simulink model "Sistemas"  (R2020b)
settings: Solver=ode15s  StartTime=0.0  StopTime=10  MaxStep=1E-2  RelTol=1e-3
libraries: fl_lib x14, nesl_utility x8, pid_lib x1
settings Model: Creator=demil  LastModifiedBy=Maibr
settings SolverCC: AlgebraicLoopSolver=LineSearch
settings DataIOCC: SaveOutput=off  SignalLogging=off  DSMLogging=off  ReturnWorkspaceOutputs=off  TimeSaveName=t
settings DebuggingCC: AlgebraicLoopMsg=none  ArtificialAlgebraicLoopMsg=none  MaxConsecutiveZCsMsg=none  ModelReferenceExtraNoncontSigs=none  OperatingPointInterfaceChecksumMismatchMsg=none

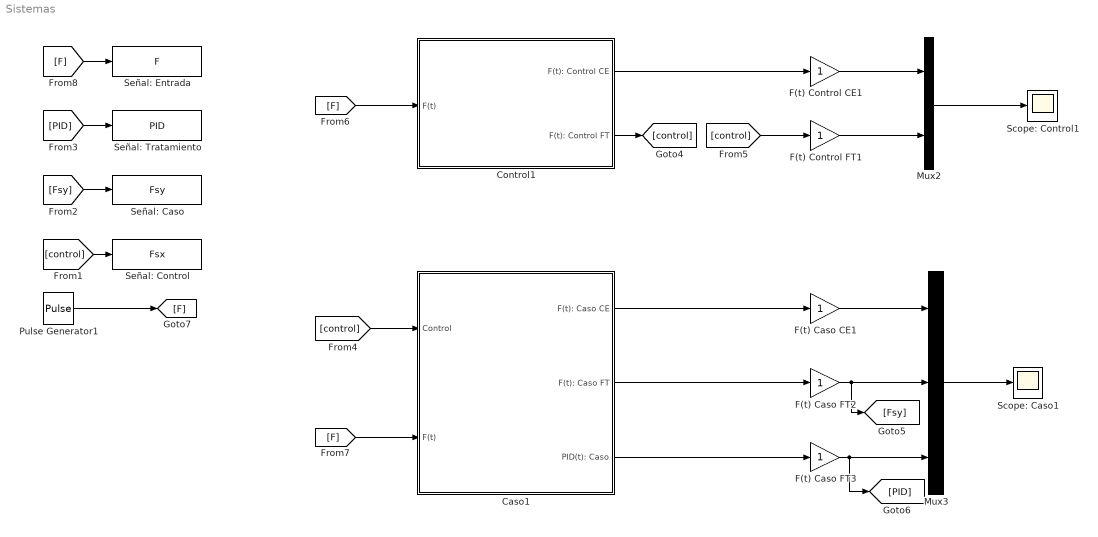
== system Sistemas ==
  Caso1 : Subsystem
  Control1 : Subsystem
  F(t) Caso CE1 : Gain
  F(t) Caso FT2 : Gain
  F(t) Caso FT3 : Gain
  F(t) Control CE1 : Gain
  F(t) Control FT1 : Gain
  Mux2 : Mux  Inputs=2
  Mux3 : Mux  Inputs=3
  Pulse Generator1 : DiscretePulseGenerator  PulseType=Time based  Period=10  PulseWidth=10  PhaseDelay=1
  Scope: Caso1 : Scope
  Scope: Control1 : Scope
  Señal: Caso : ToWorkspace  VariableName=Fsy  SampleTime=-1
  Señal: Control : ToWorkspace  VariableName=Fsx  SampleTime=-1
  Señal: Entrada : ToWorkspace  VariableName=F  SampleTime=-1
  Señal: Tratamiento : ToWorkspace  VariableName=PID  SampleTime=-1
  wires:
  [F] -> Señal: Entrada/1
  F(t) Control FT1/1 -> Mux2/2
  [PID] -> Señal: Tratamiento/1
  Caso1/3(PID(t): Caso) -> F(t) Caso FT3/1
  [F] -> Caso1/2(F(t))
  [Fsy] -> Señal: Caso/1
  [control] -> Señal: Control/1
  F(t) Caso FT3/1 -> [PID], Mux3/3
  Control1/1(F(t): Control CE) -> F(t) Control CE1/1
  [F] -> Control1/1(F(t))
  Control1/2(F(t): Control FT) -> [control]
  Caso1/2(F(t): Caso FT) -> F(t) Caso FT2/1
  F(t) Caso CE1/1 -> Mux3/1
  Pulse Generator1/1 -> [F]
  [control] -> Caso1/1(Control)
  Mux3/1 -> Scope: Caso1/1
  Caso1/1(F(t): Caso CE) -> F(t) Caso CE1/1
  F(t) Control CE1/1 -> Mux2/1
  F(t) Caso FT2/1 -> Mux3/2, [Fsy]
  [control] -> F(t) Control FT1/1
  Mux2/1 -> Scope: Control1/1

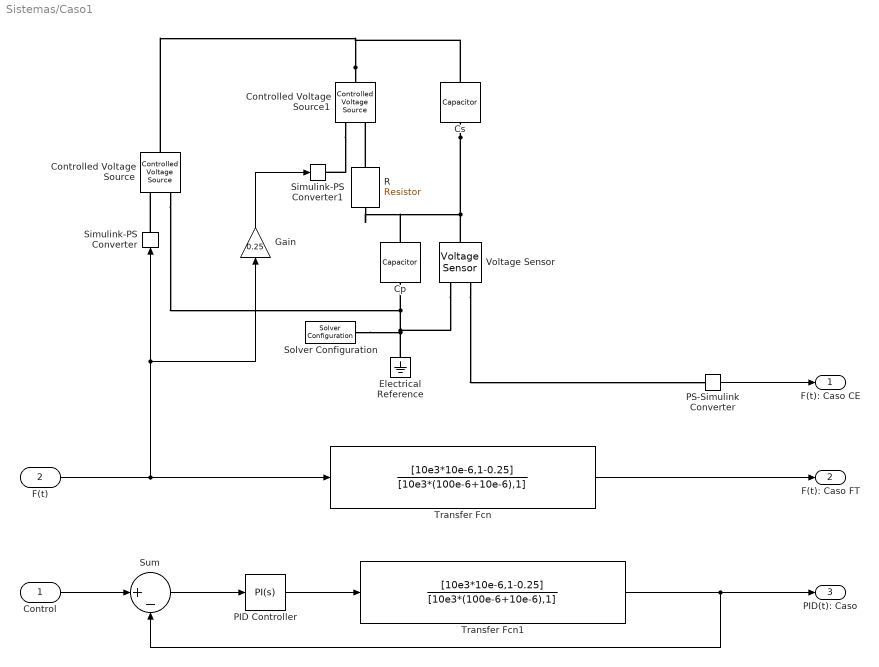
== system Sistemas/Caso1 ==
  Control : Inport
  F(t) : Inport  Port=2
  Controlled Voltage Source : fl_lib/Electrical/Electrical Sources/Controlled Voltage Source
  Controlled Voltage Source1 : fl_lib/Electrical/Electrical Sources/Controlled Voltage Source
  Cp : fl_lib/Electrical/Electrical Elements/Capacitor  c=100 uF  r=1e-6 Ohm  g=0 1/Ohm  i_specify=off  i_priority=None  i=0 A  i_nominal_specify=off  i_nominal_unit=A  i_nominal_value=1  v_specify=off  v_priority=None  v=0 V  v_nominal_specify=off  v_nominal_unit=V  v_nominal_value=1  vc_specify=off  vc_priority=High  vc=0 V  vc_nominal_specify=off  vc_nominal_unit=V  vc_nominal_value=1
  Cs : fl_lib/Electrical/Electrical Elements/Capacitor  c=10 uF  r=1e-6 Ohm  g=0 1/Ohm  i_specify=off  i_priority=None  i=0 A  i_nominal_specify=off  i_nominal_unit=A  i_nominal_value=1  v_specify=off  v_priority=None  v=0 V  v_nominal_specify=off  v_nominal_unit=V  v_nominal_value=1  vc_specify=off  vc_priority=High  vc=0 V  vc_nominal_specify=off  vc_nominal_unit=V  vc_nominal_value=1
  Electrical Reference : fl_lib/Electrical/Electrical Elements/Electrical Reference
  Gain : Gain  Gain=0.25
  PID Controller : pid_lib/PID Controller  Controller=PI  Form=Parallel  TimeDomain=Continuous-time  UseExternalTs=off  SampleTime=-1  IntegratorMethod=Forward Euler  FilterMethod=Forward Euler  ControllerParametersSource=internal  P=0.218837731319984  I=3640.74282297537  D=0  UseFilter=on  N=100  TunerSelectOption=Transfer Function Based (PID Tuner App)  InitialConditionSource=internal  InitialConditionForIntegrator=0  InitialConditionForFilter=0  DifferentiatorICPrevScaledInput=0  ExternalReset=none  TrackingMode=off  Kt=1  LimitOutput=off  SatLimitsSource=internal  UpperSaturationLimit=inf  LowerSaturationLimit=-inf  LinearizeAsGain=on  AntiWindupMode=none  Kb=1  POutMin=[]  POutMax=[]  IOutMin=[]  IOutMax=[]  DOutMin=[]  DOutMax=[]  NOutMin=[]  NOutMax=[]  SumOutMin=[]  SumOutMax=[]  SaturationOutMin=[]  SaturationOutMax=[]  PParamMin=[]  PParamMax=[]  IParamMin=[]  IParamMax=[]  DParamMin=[]  DParamMax=[]  NParamMin=[]  NParamMax=[]  KbParamMin=[]  KbParamMax=[]  KtParamMin=[]  KtParamMax=[]  KbOutMin=[]  KbOutMax=[]  KtOutMin=[]  KtOutMax=[]  IntegratorOutMin=[]  IntegratorOutMax=[]  FilterOutMin=[]  FilterOutMax=[]  SumI1OutMin=[]  SumI1OutMax=[]  SumI2OutMin=[]  SumI2OutMax=[]  SumI3OutMin=[]  SumI3OutMax=[]  SumI4OutMin=[]  SumI4OutMax=[]  SumDOutMin=[]  SumDOutMax=[]  DifferentiatorOutMin=[]  DifferentiatorOutMax=[]  FilterDiffOutCoefMin=[]  FilterDiffOutCoefMax=[]  ReciprocalOutMin=[]  ReciprocalOutMax=[]  SumDenOutMin=[]  SumDenOutMax=[]  SumNumOutMin=[]  SumNumOutMax=[]  DivideOutMin=[]  DivideOutMax=[]  UdiffTsProdOutMin=[]  UdiffTsProdOutMax=[]  NTsProdOutMin=[]  NTsProdOutMax=[]  UintegralTsProdOutMin=[]  UintegralTsProdOutMax=[]  UngainTsProdOutMin=[]  UngainTsProdOutMax=[]  IntegratorContinuousStateAttributes=''  IntegratorStateMustResolveToSignalObject=off  IntegratorRTWStateStorageClass=Auto  FilterContinuousStateAttributes=''  FilterStateMustResolveToSignalObject=off  FilterRTWStateStorageClass=Auto  ParallelPVariant=InternalParameters  IdealPVariant=Disabled  IVariant=InternalParameters  DVariant=Disabled  IntegratorVariant=Continuous  SatVariant=Disabled  AWVariant=Passthrough  PCopyVariant=Disabled  TRVariant=Disabled  FdbkBlocksVariant=Forward  IdealPFdbkVariant=Disabled  SatFdbkVariant=Disabled  DerivativeFilterVariant=Disabled  NVariant=Disabled  NCopyVariant=Disabled_SignalSpec  FilterICVariant=Disabled  IntegratorICVariant=InternalICs  ExternalResetVariant=Disabled  TRSumVariant=Passthrough  SumFdbkVariant=Disabled  SumVariant=Sum_PI  TsampFilterVariant=InternalTs  TsampNgainVariant=Passthrough  TsampIntegralVariant=Passthrough  ExternalSaturationOutDataTypeStr=Inherit: Same as second input
  PS-Simulink Converter : nesl_utility/PS-Simulink Converter  PhysicalDomain=network_engine_domain  SubClassName=ps_output  LeftPortType=input  RightPortType=output  PseudoPeriodic=off  Frequencies=[]  Unit=inherit  AffineConversion=off
  R : fl_lib/Electrical/Electrical Elements/Resistor  R=10 kOhm  i_specify=off  i_priority=None  i=0 A  i_nominal_specify=off  i_nominal_unit=A  i_nominal_value=1  v_specify=off  v_priority=None  v=0 V  v_nominal_specify=off  v_nominal_unit=V  v_nominal_value=1
  Simulink-PS Converter : nesl_utility/Simulink-PS Converter  PhysicalDomain=network_engine_domain  SubClassName=ps_input  LeftPortType=input  RightPortType=output  PseudoPeriodic=off  Frequencies=[]  NoiseDistribution=none  NoiseParameters=[]  Unit=1  AffineConversion=off  FilteringAndDerivatives=provide  SimscapeFilterOrder=1  InputFilterTimeConstant=0.001  UdotUserProvided=0
  Simulink-PS Converter1 : nesl_utility/Simulink-PS Converter  PhysicalDomain=network_engine_domain  SubClassName=ps_input  LeftPortType=input  RightPortType=output  PseudoPeriodic=off  Frequencies=[]  NoiseDistribution=none  NoiseParameters=[]  Unit=1  AffineConversion=off  FilteringAndDerivatives=provide  SimscapeFilterOrder=1  InputFilterTimeConstant=0.001  UdotUserProvided=0
  Solver Configuration : nesl_utility/Solver Configuration  PhysicalDomain=network_engine_domain  SubClassName=solver  LeftPortType=input  RightPortType=generic  Tones=[]  Harmonics=[]  SimulateNoise=off  Profile=off  UseLocalSampling=off  EnableSwitchedLinearOptims=on  FrequencyDomain=off  UseCCode=off  RelTol=0.001  AbsTol=0.001  MinStep=1e-09  ToWorkspace=off  RevertToSquareIcSolve=off  NumHomotopyIterations=100  PhasorMode=off  PhasorModeNumHarmonics=1  DoDC=off  ResidualTolerance=1e-09  UseLocalSolver=off  LocalSolverChoice=NE_BACKWARD_EULER_ADVANCER  LocalSolverSampleTime=0.001  DoFixedCost=off  MaxNonlinIter=3  MaxModeIter=2  ComputeImpulses=off  ImpulseIterations=2  LinearAlgebra=auto  EquationFormulation=NE_TIME_EF  DelaysMemoryBudget=1024  AutomaticFiltering=on  FilteringTimeConstant=0.001  PartitionStorageMethod=AS_NEEDED  PartitionMemoryBudget=1024  PartitionMethod=ROBUST
  Sum : Sum  Inputs=|+-
  Transfer Fcn : TransferFcn  Numerator=[10e3*10e-6,1-0.25]  Denominator=[10e3*(100e-6+10e-6),1]
  Transfer Fcn1 : TransferFcn  Numerator=[10e3*10e-6,1-0.25]  Denominator=[10e3*(100e-6+10e-6),1]
  Voltage Sensor : fl_lib/Electrical/Electrical Sensors/Voltage Sensor
  F(t): Caso CE : Outport
  F(t): Caso FT : Outport  Port=2
  PID(t): Caso : Outport  Port=3
  wires:
  Gain/1 -> Simulink-PS Converter1/1
  PS-Simulink Converter/1 -> F(t): Caso CE/1
  Transfer Fcn/1 -> F(t): Caso FT/1
  F(t)/1 -> Gain/1, Simulink-PS Converter/1, Transfer Fcn/1
  Control/1 -> Sum/1
  Sum/1 -> PID Controller/1
  PID Controller/1 -> Transfer Fcn1/1
  Transfer Fcn1/1 -> Sum/2, PID(t): Caso/1
  connections:
  Simulink-PS Converter/RConn1 -- Controlled Voltage Source/RConn1
  Controlled Voltage Source1/RConn1 -- Simulink-PS Converter1/RConn1
  Controlled Voltage Source1/LConn1 -- Controlled Voltage Source/LConn1 -- Cs/LConn1
  R/LConn1 -- Controlled Voltage Source1/RConn2
  Cs/RConn1 -- Voltage Sensor/LConn1 -- R/RConn1 -- Cp/LConn1
  Solver Configuration/RConn1 -- Electrical Reference/LConn1 -- Voltage Sensor/RConn2 -- Cp/RConn1 -- Controlled Voltage Source/RConn2
  Voltage Sensor/RConn1 -- PS-Simulink Converter/LConn1

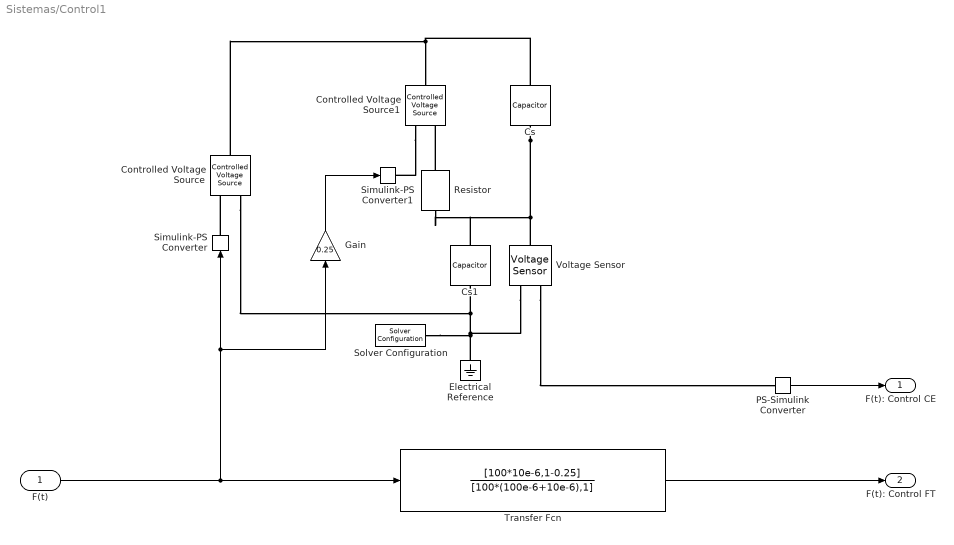
== system Sistemas/Control1 ==
  F(t) : Inport
  Controlled Voltage Source : fl_lib/Electrical/Electrical Sources/Controlled Voltage Source
  Controlled Voltage Source1 : fl_lib/Electrical/Electrical Sources/Controlled Voltage Source
  Cs : fl_lib/Electrical/Electrical Elements/Capacitor  c=10 uF  r=1e-6 Ohm  g=0 1/Ohm  i_specify=off  i_priority=None  i=0 A  i_nominal_specify=off  i_nominal_unit=A  i_nominal_value=1  v_specify=off  v_priority=None  v=0 V  v_nominal_specify=off  v_nominal_unit=V  v_nominal_value=1  vc_specify=off  vc_priority=High  vc=0 V  vc_nominal_specify=off  vc_nominal_unit=V  vc_nominal_value=1
  Cs1 : fl_lib/Electrical/Electrical Elements/Capacitor  c=100 uF  r=1e-6 Ohm  g=0 1/Ohm  i_specify=off  i_priority=None  i=0 A  i_nominal_specify=off  i_nominal_unit=A  i_nominal_value=1  v_specify=off  v_priority=None  v=0 V  v_nominal_specify=off  v_nominal_unit=V  v_nominal_value=1  vc_specify=off  vc_priority=High  vc=0 V  vc_nominal_specify=off  vc_nominal_unit=V  vc_nominal_value=1
  Electrical Reference : fl_lib/Electrical/Electrical Elements/Electrical Reference
  Gain : Gain  Gain=0.25
  PS-Simulink Converter : nesl_utility/PS-Simulink Converter  PhysicalDomain=network_engine_domain  SubClassName=ps_output  LeftPortType=input  RightPortType=output  PseudoPeriodic=off  Frequencies=[]  Unit=inherit  AffineConversion=off
  Resistor : fl_lib/Electrical/Electrical Elements/Resistor  R=100 Ohm  i_specify=off  i_priority=None  i=0 A  i_nominal_specify=off  i_nominal_unit=A  i_nominal_value=1  v_specify=off  v_priority=None  v=0 V  v_nominal_specify=off  v_nominal_unit=V  v_nominal_value=1
  Simulink-PS Converter : nesl_utility/Simulink-PS Converter  PhysicalDomain=network_engine_domain  SubClassName=ps_input  LeftPortType=input  RightPortType=output  PseudoPeriodic=off  Frequencies=[]  NoiseDistribution=none  NoiseParameters=[]  Unit=1  AffineConversion=off  FilteringAndDerivatives=provide  SimscapeFilterOrder=1  InputFilterTimeConstant=0.001  UdotUserProvided=0
  Simulink-PS Converter1 : nesl_utility/Simulink-PS Converter  PhysicalDomain=network_engine_domain  SubClassName=ps_input  LeftPortType=input  RightPortType=output  PseudoPeriodic=off  Frequencies=[]  NoiseDistribution=none  NoiseParameters=[]  Unit=1  AffineConversion=off  FilteringAndDerivatives=provide  SimscapeFilterOrder=1  InputFilterTimeConstant=0.001  UdotUserProvided=0
  Solver Configuration : nesl_utility/Solver Configuration  PhysicalDomain=network_engine_domain  SubClassName=solver  LeftPortType=input  RightPortType=generic  Tones=[]  Harmonics=[]  SimulateNoise=off  Profile=off  UseLocalSampling=off  EnableSwitchedLinearOptims=on  FrequencyDomain=off  UseCCode=off  RelTol=0.001  AbsTol=0.001  MinStep=1e-09  ToWorkspace=off  RevertToSquareIcSolve=off  NumHomotopyIterations=100  PhasorMode=off  PhasorModeNumHarmonics=1  DoDC=off  ResidualTolerance=1e-09  UseLocalSolver=off  LocalSolverChoice=NE_BACKWARD_EULER_ADVANCER  LocalSolverSampleTime=0.001  DoFixedCost=off  MaxNonlinIter=3  MaxModeIter=2  ComputeImpulses=off  ImpulseIterations=2  LinearAlgebra=auto  EquationFormulation=NE_TIME_EF  DelaysMemoryBudget=1024  AutomaticFiltering=on  FilteringTimeConstant=0.001  PartitionStorageMethod=AS_NEEDED  PartitionMemoryBudget=1024  PartitionMethod=ROBUST
  Transfer Fcn : TransferFcn  Numerator=[100*10e-6,1-0.25]  Denominator=[100*(100e-6+10e-6),1]
  Voltage Sensor : fl_lib/Electrical/Electrical Sensors/Voltage Sensor
  F(t): Control CE : Outport
  F(t): Control FT : Outport  Port=2
  wires:
  F(t)/1 -> Gain/1, Simulink-PS Converter/1, Transfer Fcn/1
  Gain/1 -> Simulink-PS Converter1/1
  PS-Simulink Converter/1 -> F(t): Control CE/1
  Transfer Fcn/1 -> F(t): Control FT/1
  connections:
  Simulink-PS Converter/RConn1 -- Controlled Voltage Source/RConn1
  Controlled Voltage Source1/RConn1 -- Simulink-PS Converter1/RConn1
  Cs/LConn1 -- Controlled Voltage Source/LConn1 -- Controlled Voltage Source1/LConn1
  Resistor/LConn1 -- Controlled Voltage Source1/RConn2
  Cs/RConn1 -- Voltage Sensor/LConn1 -- Resistor/RConn1 -- Cs1/LConn1
  Solver Configuration/RConn1 -- Electrical Reference/LConn1 -- Voltage Sensor/RConn2 -- Cs1/RConn1 -- Controlled Voltage Source/RConn2
  Voltage Sensor/RConn1 -- PS-Simulink Converter/LConn1
